simulink model "2DOF_linear_tire"  (R2024a)
settings: Solver=ode1  StartTime=0.0  StopTime=10  FixedStep=0.001  RelTol=1e-3
PostLoadFcn:
  | , if any(exist('dsrtsu_mdlpostloadfcn', 'file') == [2, 3, 6]), try dsrtsu_mdlpostloadfcn('Execute', bdroot); catch fprintf('Error in PostLoadFcn (dsrtsu_mdlpostloadfcn) for model "%s":\n %s\n', bdroot, lasterr); end, end,
InitFcn:
  | , if any(exist('rtifpga_mdlclblib', 'file') ~= 0), rtifpga_mdlclblib('Init', bdroot); end,
values from neighbouring files (symbols this model uses):
  Ap = [0, 1, 0, 0 ... (first row only)    [init_parameters.m]
  As = Ap    [init_parameters.m]
  Bp = [0 ... (first row only)    [init_parameters.m]
  Bs = [0, 0, 0 ... (first row only)    [init_parameters.m]
  Cp = eye(4)    [init_parameters.m]
  Cs = Cp    [init_parameters.m]
  Dp = zeros(4, 1)    [init_parameters.m]
  Ds = zeros(4, 3)    [init_parameters.m]
  K = lqr(As, B_control, Q, R)    [init_parameters.m]
Description:
  | Standard RTI1401 template.
  | Supported MATLAB version:  R2024a.
settings Model: Tag=RTI1401  DSRTSU_INTERNAL_RTI_VER=640  DSRTSU_INTERNAL_RTI_TYPE=rti1401  RTICANMMDATA=struct('GeneralSetupData',struct('modelroot','C:\Users\VM-User\Desktop\MigrationScripts','generalsettings',struct('filesettings',struct('destfolder',struct('Name','RTICANMM_FILES','Check',1),'buildfolder',struct('Name','.','Check',1),'AbsDestfolder',struct('Name','C:\Users\VM-User\Desktop\MigrationScripts\RTICANMM_FILES'),'AbsBuildfolder',struct('Name','C:\Users\VM-User\Desktop\MigrationScripts'))),'options',struct('addpaths',1,'rmpaths',1,'addtrcexclusion',true,'cannavigator',struct('checkmonitoring',0),'show_usrtrc',0,'use_usrtrc',0),'advanced',struct('options',ones(1,100)),'MPSetup',{{}},'RTI',struct('Type','RTI1401','Ver','7.17','Date','02-Nov-2021'),'modelname','','block','untitled'))  DSRTSU_INTERNAL_RTIFPGA=210  DSRTSU_INTERNAL_RTISTBM_VER=24.1  Creator=ivanv  LastModifiedBy=ivanv
settings SolverCC: AlgebraicLoopSolver=TrustRegion
settings DataIOCC: ReturnWorkspaceOutputs=off
settings OptimizationCC: BlockReduction=off  OptimizeBlockIOStorage=off  BufferReuse=off  ReuseModelBlockBuffer=off  GlobalBufferReuse=off  ExpressionFolding=off  LocalBlockOutputs=off  OptimizeDataStoreBuffers=off  BusAssignmentInplaceUpdate=off
settings DebuggingCC: UnconnectedInputMsg=warning  UnconnectedOutputMsg=warning  UnconnectedLineMsg=warning  PregeneratedLibrarySubsystemCodeDiagnostic=none  ArithmeticOperatorsInVariantConditions=warning
settings HardwareCC: ProdBitPerPointer=32  ProdBitPerSizeT=32  ProdBitPerPtrDiffT=32  ProdLargestAtomicInteger=Integer  ProdEndianess=BigEndian  ProdWordSize=32  ProdLongLongMode=on  ProdHWDeviceType=Custom Processor->Custom  TargetIntDivRoundTo=Zero  TargetEndianess=BigEndian  TargetHWDeviceType=Custom Processor->Custom
settings ModelReferenceCC: EnableRefExpFcnMdlSchedulingChecks=on  EnableParallelModelReferenceBuilds=on  ParallelModelReferenceMATLABWorkerInit=Load Top Model
settings SFSimCC: SimUseLocalCustomCode=off  MATLABDynamicMemAlloc=off  CustomCodeUndefinedFunction=UseInterfaceOnly
settings RTWCC: Description=dSPACE DS1401 Hardware Platform  SystemTargetFile=rti1401.tlc  MakeCommand=make_rti  TemplateMakefile=rti1401.tmf  RTWUseLocalCustomCode=off  GPUComputeCapability=3.5  DLArmComputeVersion=19.05
settings CodeAppCC: StateflowObjectComments=on
settings STFCustomTargetCC: TargetLangStandard=C89/C90 (ANSI)  ParMdlRefBuildCompliant=on  MatFileLogging=on  GRTInterface=off  UseToolchainInfoCompliant=off  SystemTargetFile=rti1401.tlc
settings GRTTargetCC: TargetLangStandard=C89/C90 (ANSI)  CompOptLevelCompliant=off  ConcurrentExecutionCompliant=off  CombineOutputUpdateFcns=off  CPPClassGenCompliant=off  UseToolchainInfoCompliant=off
settings ConfigComp: CovMetricSettings=dswe

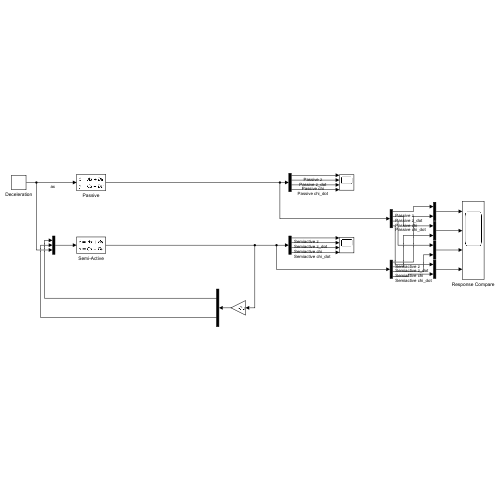
[thumbnail: Simulink's stored preview of the top-level diagram]
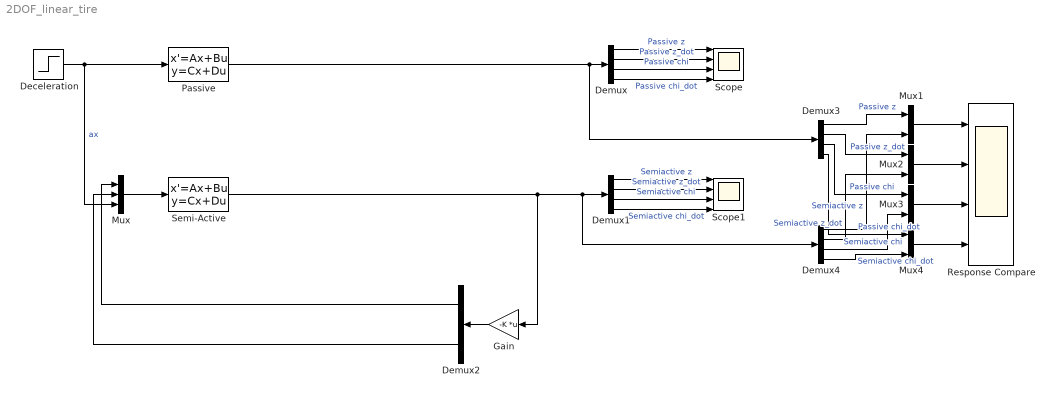
== system 2DOF_linear_tire ==
  Deceleration : Step  After=8  SampleTime=0
  Demux{,1,3..4} (4 alike) : Demux
  Demux2 : Demux  Outputs=2
  Gain : Gain  Gain=-K  Multiplication=Matrix(K*u)
  Mux : Mux  Inputs=3
  Mux{1..4} (4 alike) : Mux  Inputs=2
  Passive : StateSpace  A=Ap  B=Bp  C=Cp  D=Dp  InitialCondition=0
  Response Compare : Scope  NumInputPorts=4
  Scope : Scope  NumInputPorts=4
  Scope1 : Scope  NumInputPorts=4
  Semi-Active : StateSpace  A=As  B=Bs  C=Cs  D=Ds  InitialCondition=0
  wires:
  Deceleration/1 -> Mux/3, Passive/1  "ax"
  Passive/1 -> Demux3/1, Demux/1
  Demux/1 -> Scope/1  "Passive z"
  Demux/2 -> Scope/2  "Passive z_dot"
  Demux/3 -> Scope/3  "Passive chi"
  Demux/4 -> Scope/4  "Passive chi_dot"
  Mux/1 -> Semi-Active/1
  Semi-Active/1 -> Demux4/1, Demux1/1, Gain/1
  Demux1/1 -> Scope1/1  "Semiactive z"
  Demux1/2 -> Scope1/2  "Semiactive z_dot"
  Demux1/4 -> Scope1/4  "Semiactive chi_dot"
  Demux1/3 -> Scope1/3  "Semiactive chi"
  Mux1/1 -> Response Compare/1
  Mux2/1 -> Response Compare/2
  Mux3/1 -> Response Compare/3
  Mux4/1 -> Response Compare/4
  Demux3/1 -> Mux1/1  "Passive z"
  Demux4/1 -> Mux1/2  "Semiactive z"
  Demux3/2 -> Mux2/1  "Passive z_dot"
  Demux4/2 -> Mux2/2  "Semiactive z_dot"
  Demux3/3 -> Mux3/1  "Passive chi"
  Demux4/3 -> Mux3/2  "Semiactive chi"
  Demux3/4 -> Mux4/1  "Passive chi_dot"
  Demux4/4 -> Mux4/2  "Semiactive chi_dot"
  Gain/1 -> Demux2/1
  Demux2/1 -> Mux/1
  Demux2/2 -> Mux/2
